simulink model "biogass"  (R2025a)
settings: Solver=VariableStepAuto  StartTime=0.0  StopTime=10.0  RelTol=1e-3
libraries: spsGroundLib x4, spsCurrentMeasurementLib x2, simulink x2, spsControlledVoltageSourceLib x1, spsPVArrayLib x1, spsSeriesRLCBranchLib x1, spsVoltageMeasurementLib x1, sps_lib x1
settings Model: Creator=Rishitha  LastModifiedBy=Rishitha

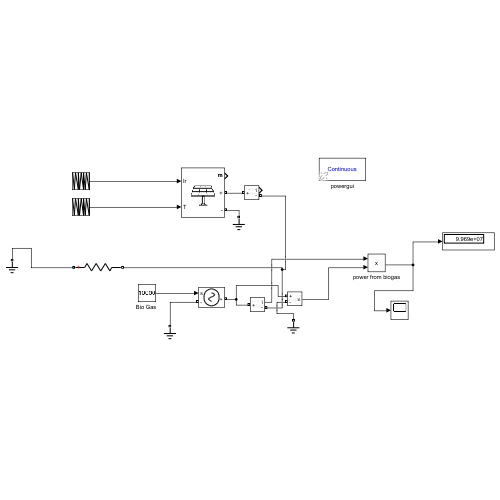
[thumbnail: Simulink's stored preview of the top-level diagram]
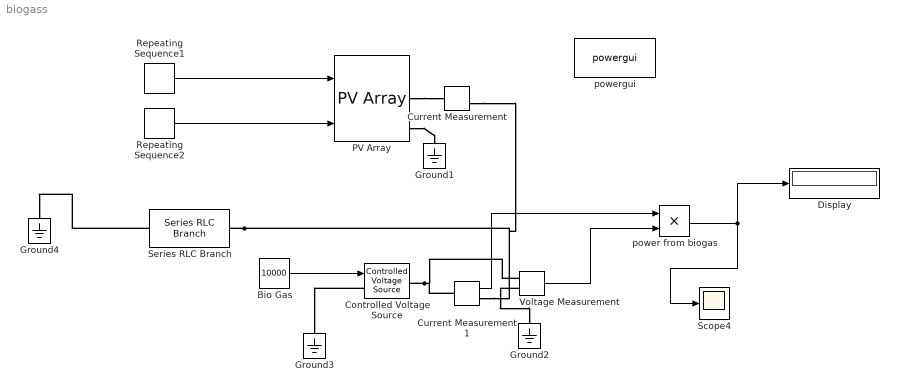
== system biogass ==
  "Bio Gas " : Constant  Value=10000
  Controlled Voltage Source : spsControlledVoltageSourceLib/Controlled Voltage Source  Initialize=on  Source_Type=AC  Amplitude=0  Phase=0  Frequency=0  Measurements=None
  Current Measurement : spsCurrentMeasurementLib/Current Measurement  PhasorSimulation=off  OutputType=Complex  PSBequivalent=0
  Current Measurement1 : spsCurrentMeasurementLib/Current Measurement  PhasorSimulation=off  OutputType=Complex  PSBequivalent=0
  Display : Display
  Ground{1..4} (4 alike) : spsGroundLib/Ground  LConnTagsString=a
  PV Array : spsPVArrayLib/PV Array  Npar=4  Nser=10  PlotType=array @ 1000 W/m2 & specified temperatures  S_vec="[ 1000  500  100 ]"  Temp_C_vec="[ 45 25  ]"  ModuleName=Trina Solar TSM-275PA14  PlotWhenSelected=off  Pm=275.328  Ncell=72  Voc=44.4  Isc=8.39  Vm=35.85  Im=7.68  beta_Voc_pc=-0.36  alpha_Isc_pc=0.06  beta_Voc=-0.15984  alpha_Isc=0.005034  IL=8.4178  I0=2.8124e-10  nI=0.99686  Rsh=121.4327  Rs=0.40249  RobustModel=off  RobustCellTemperature=313.3991  BAL=off  Tc=1e-6  Tfilter=5e-5
  Repeating Sequence1 : simulink/Sources/Repeating Sequence  rep_seq_t=[0 7 12 24]  rep_seq_y=[1000 200 1000 200]
  Repeating Sequence2 : simulink/Sources/Repeating Sequence  rep_seq_t=[0 7 12 24]  rep_seq_y=[30 20 30 20]
  Scope4 : Scope
      settings: ActiveDisplayYMinimum=8.3847902797287971E+7  ActiveDisplayYMaximum=2.2018453416925645E+8  DataLoggingVariableName=ScopeData3
  Series RLC Branch : spsSeriesRLCBranchLib/Series RLC Branch  LConnTagsString=__new0  RConnTagsString=__new0  BranchType=R  Resistance=1  Inductance=1e-3  SetiL0=off  InitialCurrent=0  Capacitance=1e-6  Setx0=off  InitialVoltage=0  Measurements=None
  Voltage Measurement : spsVoltageMeasurementLib/Voltage Measurement  PhasorSimulation=off  OutputType=Complex  PSBequivalent=0
  power from biogas : Product
  powergui : sps_lib/powergui  Priority=1  SimulationMode=Continuous  SampleTime=50e-6  frequency=60  Iterations=50  frequencyindice=0  Pbase=100e6  ErrMax=1e-4  UnitsV=kV  UnitsW=MW  buscounter=0  FunctionMessages=off  echomessages=off  EnableUseOfTLC=off  CurrentSourceSwitches=off  DisableSnubberDevices=off  DisableRonSwitches=off  DisableVfSwitches=off  DisplayEquations=off  AutomaticDiscreteSolvers=off  SolverType=Tustin/Backward Euler (TBE)  Interpol=off  ExternalGateDelay=off  methode=off  Ts=100  x0status=blocks  SPID=on  SwTol=0  HookPort=off  NonlinearTolerance=1e-4  nMaxIteration=100  ContinueOnMaxIteration=off  RestoreLinks=warning  ResistiveCurrentMeasurement=off  Frange=[0:2:500]  Ylog=off  Xlog=on  ShowGrid=off  save=off  variable=ZData  structure=0  ZoomFFT=off  StartTime=0.0  cycles=1  DisplayStyle=1  fundamental=60  FreqAxis=off  MaxFrequency=1000  frequencyindicesteady=1  RmsSteady=1  display=off
  wires:
  Voltage Measurement/1 -> power from biogas/2
  Current Measurement1/1 -> power from biogas/1
  "Bio Gas "/1 -> Controlled Voltage Source/1
  power from biogas/1 -> Display/1, Scope4/1
  Repeating Sequence2/1 -> PV Array/2
  Repeating Sequence1/1 -> PV Array/1
  connections:
  Series RLC Branch/RConn1 -- Current Measurement/RConn1 -- Current Measurement1/RConn1
  Controlled Voltage Source/RConn1 -- Current Measurement1/LConn1 -- Voltage Measurement/LConn1
  Voltage Measurement/LConn2 -- Ground2/LConn1
  Controlled Voltage Source/LConn1 -- Ground3/LConn1
  Series RLC Branch/LConn1 -- Ground4/LConn1
  PV Array/RConn1 -- Current Measurement/LConn1
  PV Array/RConn2 -- Ground1/LConn1
